simulink model "ParameterEstimation_Testbench"  (R2025b)
settings: Solver=ode23t  StartTime=0.0  StopTime=3  MaxStep=0.0001  RelTol=1e-3
values from neighbouring files (symbols this model uses):
  B_load = 0.02    [init_estimation.m]
  J_load = 0.05    [init_estimation.m]
  Ts_exp = 0.002    [init_estimation.m]
settings Model: Creator=Compu  LastModifiedBy=Compu

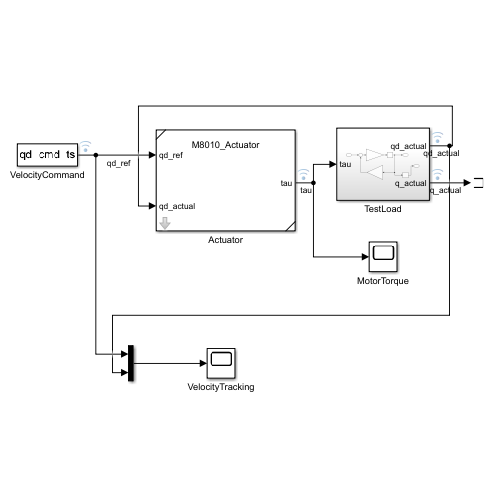
[thumbnail: Simulink's stored preview of the top-level diagram]
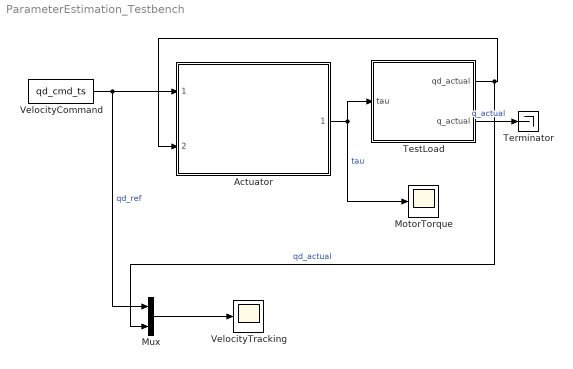
== system ParameterEstimation_Testbench ==
  Actuator : Subsystem  ReferencedSubsystem=M8010_Actuator  VelKp=0.00076207895  VelKi=0.0015241579
  MotorTorque : Scope
      settings: ActiveDisplayYMinimum=-0.21255412605172441  ActiveDisplayYMaximum=0.21634706234906778
  Mux : Mux  Inputs=2
  Terminator : Terminator
  TestLoad : Subsystem
  VelocityCommand : FromWorkspace  VariableName=qd_cmd_ts  SampleTime=Ts_exp  Interpolate=off  OutputAfterFinalValue=Holding final value
  VelocityTracking : Scope
      settings: ActiveDisplayYMinimum=-0.0529503529718834  ActiveDisplayYMaximum=0.25354473688738033
  wires:
  VelocityCommand/1 -> Mux/1, Actuator/1  "qd_ref"
  Actuator/1 -> MotorTorque/1, TestLoad/1(tau)  "tau"
  TestLoad/1(qd_actual) -> Mux/2, Actuator/2  "qd_actual"
  Mux/1 -> VelocityTracking/1
  TestLoad/2(q_actual) -> Terminator/1  "q_actual"

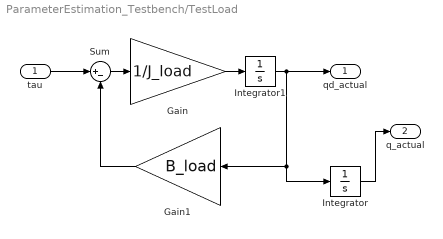
== system ParameterEstimation_Testbench/TestLoad ==
  tau : Inport
  Gain : Gain  Gain=1/J_load
  Gain1 : Gain  Gain=B_load
  Integrator : Integrator
  Integrator1 : Integrator
  Sum : Sum  Inputs=|+-
  qd_actual : Outport
  q_actual : Outport  Port=2
  wires:
  tau/1 -> Sum/1
  Gain1/1 -> Sum/2
  Sum/1 -> Gain/1
  Gain/1 -> Integrator1/1
  Integrator1/1 -> Integrator/1, Gain1/1, qd_actual/1
  Integrator/1 -> q_actual/1
